simulink model "planta_codesys_opc"  (R2025b)
settings: Solver=FixedStepAuto  StartTime=0.0  StopTime=inf  FixedStep=Ts2  RelTol=1e-3
values from neighbouring files (symbols this model uses):
  ah_max = 0.75    [init_plant_parameters.m]
  at_max = 0.80    (= 0.8)    [init_plant_parameters.m]
  bcx = 1.0e6    (= 1000000)    [init_plant_parameters.m]
  bcy = 10.0e6    (= 10000000)    [init_plant_parameters.m]
  bh_eq = bhm+bhd/ih^2    (= 18.0165289256)    [init_plant_parameters.m]
  bhb = 100e6    (= 100000000)    [init_plant_parameters.m]
  bhEb = 2.2e9    (= 2200000000)    [init_plant_parameters.m]
  bhwu = 150    [init_plant_parameters.m]
  bt = 90.0    (= 90)    [init_plant_parameters.m]
  bt_eq = btm+btd/it^2    (= 6.002)    [init_plant_parameters.m]
  btb = 5.0e6    (= 5000000)    [init_plant_parameters.m]
  btw = 3.0e3    (= 3000)    [init_plant_parameters.m]
  g = 9.80665    [init_plant_parameters.m]
  Hc = 2.59    [init_plant_parameters.m]
  ih = 22.0    (= 22)    [init_plant_parameters.m]
  it = 30.0    (= 30)    [init_plant_parameters.m]
  Jh_eq = Jhm_hb+Jhd_hEb/ih^2    (= 37.8512396694)    [init_plant_parameters.m]
  Jt_eq = Jtm_tb+Jtd/it^2    (= 8.33333333333)    [init_plant_parameters.m]
  k_i_c = abs(polos_obs_c)^3    [init_plant_parameters.m]
  k_i_h = abs(polos_obs_h)^3    [init_plant_parameters.m]
  k_omega_c = 3 * abs(polos_obs_c)^2    [init_plant_parameters.m]
  k_omega_h = 3 * abs(polos_obs_h)^2-k_tita_h*bh_eq/Jh_eq    [init_plant_parameters.m]
  k_tita_c = 3 * abs(polos_obs_c)    [init_plant_parameters.m]
  k_tita_h = 3 * abs(polos_obs_h)-bh_eq/Jh_eq    [init_plant_parameters.m]
  Kcy = 1.8e9    (= 1800000000)    [init_plant_parameters.m]
  khwu = 236e6    (= 236000000)    [init_plant_parameters.m]
  Ki_c = (wn_t^2*Mt)/Kf    (= 320)    [init_plant_parameters.m]
  Ki_i = (wn_h^2)*Jh_eq    (= 2422.47933884)    [init_plant_parameters.m]
  Kp_c = (2*zitta_t*wn_t*Mt)/Kf    (= 1120)    [init_plant_parameters.m]
  Kp_i = 2*zitta_h*wn_h*Jh_eq    (= 1211.23966942)    [init_plant_parameters.m]
  Ktw = 480e3    (= 480000)    [init_plant_parameters.m]
  Lh0 = 110    [init_plant_parameters.m]
  lh_0 = Yt0-yh_0    (= 7)    [init_plant_parameters.m]
  Mc_max = 50000    [init_plant_parameters.m]
  Mc_min = 2000    [init_plant_parameters.m]
  Ms = 15000    [init_plant_parameters.m]
  Mt = 30000    [init_plant_parameters.m]
  rhd = 0.75    [init_plant_parameters.m]
  rtd = 0.50    (= 0.5)    [init_plant_parameters.m]
  tau_hm = Ts2    (= 0.001)    [init_plant_parameters.m]
  tau_tm = Ts2    (= 0.001)    [init_plant_parameters.m]
  Thb_Max = 50e3    (= 50000)    [init_plant_parameters.m]
  ThEb_Max = 1.1e6    (= 1100000)    [init_plant_parameters.m]
  Thm_0 = 0    [init_plant_parameters.m]
  Thm_Max = 20e3    (= 20000)    [init_plant_parameters.m]
  titahm_0 = yl_0/(rhd/(2*ih))    (= 2228.19975108)    [init_plant_parameters.m]
  titatm_0 = xtd_0/(rtd/it)    (= 300)    [init_plant_parameters.m]
  Ts0 = 0.02    [init_plant_parameters.m]
  Ts1 = 0.02    [init_plant_parameters.m]
  Ttb_Max = 5.0e3    (= 5000)    [init_plant_parameters.m]
  Ttm_0 = 0    [init_plant_parameters.m]
  Ttm_Max = 4.0e3    (= 4000)    [init_plant_parameters.m]
  vh_0 = 0    [init_plant_parameters.m]
  vh_max = 3    [init_plant_parameters.m]
  vh_nom = 1.5    [init_plant_parameters.m]
  vt_0 = 0    [init_plant_parameters.m]
  vt_max = 4.0    (= 4)    [init_plant_parameters.m]
  Wc = 2.44    [init_plant_parameters.m]
  xl_0 = 5    [init_plant_parameters.m]
  xt_0 = 5    [init_plant_parameters.m]
  xt_max = 50.0    (= 50)    [init_plant_parameters.m]
  xt_min = -30.0    (= -30)    [init_plant_parameters.m]
  xtd_0 = xt_0    (= 5)    [init_plant_parameters.m]
  yh_max = 40    [init_plant_parameters.m]
  yh_min = -20    [init_plant_parameters.m]
  yl_0 = Yt0 - l_0    (= 37.9806775752)    [init_plant_parameters.m]
  Yt0 = 45.0    (= 45)    [init_plant_parameters.m]
  zitta = 0.5    [init_plant_parameters.m]
undefined symbols (not defined in the file or in its folder): DiscIntNeverNeededParam
libraries: opcualib x6, sl3dlib x1, simulink_extras x1, dspnetwork x1
(part 2 of 2)

== system planta_codesys_opc/Subsystem2/Observador de estado ==
  Ttm_ref : Inport
  tita_tm_enc : Inport  Port=2
  Delay One Step1 : Delay  Commented=through  DelayLength=1  InitialCondition=xtd_0
  Discrete-Time Integrator : DiscreteIntegrator  SampleTime=-1  ICPrevOutput=DiscIntNeverNeededParam  ICPrevScaledInput=DiscIntNeverNeededParam
  Discrete-Time Integrator1 : DiscreteIntegrator  InitialCondition=titatm_0  SampleTime=-1  ICPrevOutput=DiscIntNeverNeededParam  ICPrevScaledInput=DiscIntNeverNeededParam
  Discrete-Time Integrator2 : DiscreteIntegrator  SampleTime=-1  ICPrevOutput=DiscIntNeverNeededParam  ICPrevScaledInput=DiscIntNeverNeededParam
  Gain : Gain  Gain=1/Jt_eq
  Gain1 : Gain  Gain=k_omega_c
  Gain2 : Gain  Gain=k_tita_c
  Gain3 : Gain  Gain=k_i_c
  Gain4 : Gain  Gain=rtd/it
  Sum4 : Sum  Inputs=|++
  Sum5 : Sum  Inputs=|++
  Sum6 : Sum  Inputs=+-|
  Sum7 : Sum  Inputs=|++
  vt_obs : Outport
  wires:
  Discrete-Time Integrator/1 -> Sum5/1
  Sum4/1 -> Discrete-Time Integrator/1
  tita_tm_enc/1 -> Delay One Step1/1
  Discrete-Time Integrator2/1 -> Gain3/1
  Gain1/1 -> Sum4/2
  Sum6/1 -> Discrete-Time Integrator2/1, Gain1/1, Gain2/1
  Discrete-Time Integrator1/1 -> Sum6/2
  Sum7/1 -> Sum4/1
  Gain3/1 -> Sum7/2
  Gain/1 -> Sum7/1
  Gain2/1 -> Sum5/2
  Ttm_ref/1 -> Gain/1
  Sum5/1 -> Gain4/1, Discrete-Time Integrator1/1
  Delay One Step1/1 -> Sum6/1
  Gain4/1 -> vt_obs/1

== system planta_codesys_opc/Subsystem/Carro/Subsystem ==
  BRK_t : Inport
  w_tm : Inport  Port=2
  Constant : Constant  Value=0
  Gain1 : Gain  Gain=-Ttb_Max
  Gain8 : Gain  Gain=btb
  Switch : Switch  Criteria=u2 > Threshold  SaturateOnIntegerOverflow=off  InputSameDT=off
  Tanh : Trigonometry  Operator=tanh
  T_tb : Outport
  wires:
  Constant/1 -> Switch/1
  BRK_t/1 -> Switch/2
  Switch/1 -> T_tb/1  "T_tb"
  w_tm/1 -> Gain8/1
  Gain8/1 -> Tanh/1
  Tanh/1 -> Gain1/1
  Gain1/1 -> Switch/3

== system planta_codesys_opc/Subsystem/Subsystem2/Subsystem ==
  T_tm* : Inport
  Constant : Constant  Value=Ttm_Max
  Constant1 : Constant  Value=-Ttm_Max
  Gain : Gain  Gain=1/tau_tm
  Integrator : Integrator
  Max : MinMax  Function=max  Inputs=2
  Min : MinMax  Inputs=2
  Sum : Sum  Inputs=|+-
  Zero-Order Hold : ZeroOrderHold  SampleTime=tau_tm
  T_tm : Outport
  wires:
  Min/1 -> Sum/1
  Gain/1 -> Integrator/1
  Sum/1 -> Gain/1
  Integrator/1 -> Sum/2, T_tm/1
  Max/1 -> Min/2
  Constant/1 -> Min/1
  Constant1/1 -> Max/1
  T_tm*/1 -> Zero-Order Hold/1
  Zero-Order Hold/1 -> Max/2

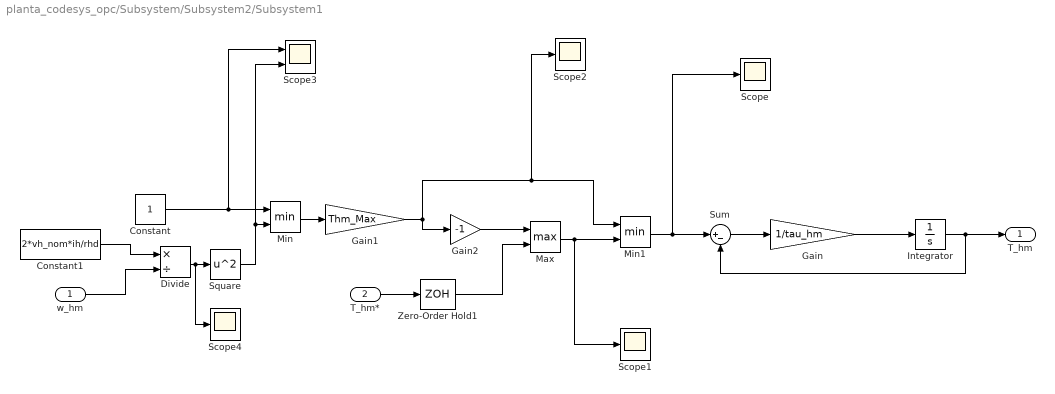
== system planta_codesys_opc/Subsystem/Subsystem2/Subsystem1 ==
  w_hm : Inport
  T_hm* : Inport  Port=2
  Constant : Constant
  Constant1 : Constant  Value=2*vh_nom*ih/rhd
  Divide : Product  Inputs=*/
  Gain : Gain  Gain=1/tau_hm
  Gain1 : Gain  Gain=Thm_Max
  Gain2 : Gain  Gain=-1
  Integrator : Integrator
  Max : MinMax  Function=max  Inputs=2
  Min : MinMax  Inputs=2
  Min1 : MinMax  Inputs=2
  Scope{,1..2,4} (4 alike) : Scope
      Scope settings: ActiveDisplayYMinimum=-2500  ActiveDisplayYMaximum=22500  DataLoggingVariableName=ScopeData3
      Scope1 settings: ActiveDisplayYMinimum=-2500  ActiveDisplayYMaximum=22500  DataLoggingVariableName=ScopeData4
      Scope2 settings: ActiveDisplayYMinimum=481.45655  ActiveDisplayYMaximum=22168.72705  DataLoggingVariableName=ScopeData5
      Scope4 settings: ActiveDisplayYMinimum=-0.06596  ActiveDisplayYMaximum=-0.00953  DataLoggingVariableName=ScopeData7
  Scope3 : Scope  NumInputPorts=2
      settings: ActiveDisplayYMinimum=-9.1717430786370772E+28  ActiveDisplayYMaximum=8.25456877077337E+29  DataLoggingVariableName=ScopeData6
  Square : Math  Operator=square
  Sum : Sum  Inputs=|+-
  Zero-Order Hold1 : ZeroOrderHold  SampleTime=tau_hm
  T_hm : Outport
  wires:
  Sum/1 -> Gain/1
  Gain/1 -> Integrator/1
  Integrator/1 -> Sum/2, T_hm/1
  Constant/1 -> Scope3/1, Min/1
  w_hm/1 -> Divide/2
  Constant1/1 -> Divide/1
  Divide/1 -> Scope4/1, Square/1
  Square/1 -> Scope3/2, Min/2
  Min/1 -> Gain1/1
  Gain1/1 -> Scope2/1, Min1/1, Gain2/1
  T_hm*/1 -> Zero-Order Hold1/1
  Gain2/1 -> Max/1
  Max/1 -> Scope1/1, Min1/2
  Min1/1 -> Scope/1, Sum/1
  Zero-Order Hold1/1 -> Max/2

== system planta_codesys_opc/Subsystem/accionamiento izaje/brake izaje ==
  w_hm : Inport
  BRK_h : Inport  Port=2
  Constant : Constant  Value=0
  Gain : Gain  Gain=bhb
  Gain1 : Gain  Gain=-Thb_Max
  Switch : Switch  Criteria=u2 > Threshold  SaturateOnIntegerOverflow=off  InputSameDT=off
  Tanh : Trigonometry  Operator=tanh
  T_hb : Outport
  wires:
  Switch/1 -> T_hb/1
  Constant/1 -> Switch/1
  BRK_h/1 -> Switch/2
  w_hm/1 -> Gain/1
  Gain/1 -> Tanh/1
  Tanh/1 -> Gain1/1
  Gain1/1 -> Switch/3

== system planta_codesys_opc/Subsystem/accionamiento izaje/brake izaje emergencia ==
  w_hd : Inport
  BRK_hE : Inport  Port=2
  Constant : Constant  Value=0
  Gain : Gain  Gain=bhEb
  Gain1 : Gain  Gain=-ThEb_Max
  Switch : Switch  Criteria=u2 > Threshold  SaturateOnIntegerOverflow=off  InputSameDT=off
  Tanh : Trigonometry  Operator=tanh
  T_hEb : Outport
  wires:
  Tanh/1 -> Gain1/1
  Gain/1 -> Tanh/1
  Constant/1 -> Switch/1
  w_hd/1 -> Gain/1
  Switch/1 -> T_hEb/1
  BRK_hE/1 -> Switch/2
  Gain1/1 -> Switch/3

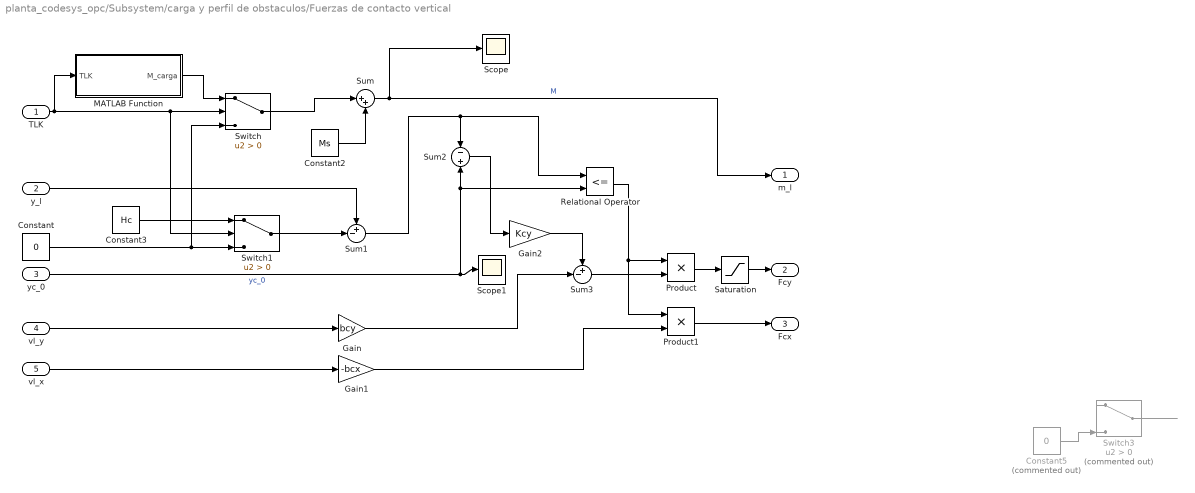
== system planta_codesys_opc/Subsystem/carga y perfil de obstaculos/Fuerzas de contacto vertical ==
  TLK : Inport
  y_l : Inport  Port=2
  yc_0 : Inport  Port=3
  vl_y : Inport  Port=4
  vl_x : Inport  Port=5
  Constant : Constant  Value=0
  Constant2 : Constant  Value=Ms
  Constant3 : Constant  Value=Hc
  Constant5 : Constant  Commented=on  Value=0
  Gain : Gain  Gain=bcy
  Gain1 : Gain  Gain=-bcx
  Gain2 : Gain  Gain=Kcy
  MATLAB Function : MATLAB Function  TreatAsAtomicUnit=on
  Product : Product
  Product1 : Product
  Relational Operator : RelationalOperator  Operator=<=  OutDataTypeStr=boolean  RndMeth=Simplest  InputSameDT=off
  Saturation : Saturate  UpperLimit=inf  LowerLimit=0
  Scope : Scope
      settings: ActiveDisplayYMinimum=-30040.049311756404  ActiveDisplayYMaximum=65258.780060315854  DataLoggingVariableName=ScopeData31
  Scope1 : Scope
      settings: ActiveDisplayYMinimum=12.776564460216019  ActiveDisplayYMaximum=15.5369149188378  DataLoggingVariableName=ScopeData32
  Sum : Sum  Inputs=|++
  Sum1 : Sum  Inputs=+-|
  Sum2 : Sum  Inputs=-|+
  Sum3 : Sum  Inputs=+-|
  Switch : Switch  Criteria=u2 > Threshold  SaturateOnIntegerOverflow=off  InputSameDT=off
  Switch1 : Switch  Criteria=u2 > Threshold  SaturateOnIntegerOverflow=off  InputSameDT=off
  Switch3 : Switch  Commented=on  Criteria=u2 > Threshold  SaturateOnIntegerOverflow=off  InputSameDT=off
  m_l : Outport
  Fcy : Outport  Port=2
  Fcx : Outport  Port=3
  wires:
  MATLAB Function/1(M_carga) -> Switch/1
  TLK/1 -> MATLAB Function/1(TLK), Switch1/2, Switch/2
  Constant/1 -> Switch1/3, Switch/3
  Constant3/1 -> Switch1/1
  Switch/1 -> Sum/1
  Sum/1 -> Scope/1, m_l/1  "M"
  Constant2/1 -> Sum/2
  Switch1/1 -> Sum1/2
  y_l/1 -> Sum1/1
  Sum1/1 -> Relational Operator/1, Sum2/1
  yc_0/1 -> Scope1/1, Sum2/2, Relational Operator/2  "yc_0"
  Sum2/1 -> Gain2/1
  Gain2/1 -> Sum3/1
  Relational Operator/1 -> Product1/1, Product/1
  Product1/1 -> Fcx/1
  Gain/1 -> Sum3/2
  vl_y/1 -> Gain/1
  vl_x/1 -> Gain1/1
  Gain1/1 -> Product1/2
  Sum3/1 -> Product/2
  Constant5/1 -> Switch3/3
  Switch3/1 -> ?
  ? -> Switch3/1, Switch3/2
  Product/1 -> Saturation/1
  Saturation/1 -> Fcy/1

== matlab function planta_codesys_opc/Subsystem/carga y perfil de obstaculos/MATLAB Function ==
  data: y0_array input; yc0_xt output; index input
function yc0_xt= calcula_y0(y0_array,index)
index = floor(index)+1;
index = min(max(index,1),33);
yc0_xt = y0_array(index);

== matlab function planta_codesys_opc/Subsystem/carga y perfil de obstaculos/Fuerzas de contacto vertical/MATLAB Function ==
  settings: updateMethod=DISCRETE
  data: TLK input; M_carga output; Mc_min parameter; Mc_max parameter
function M_carga = Masa_Aleatoria(TLK, Mc_min, Mc_max)
    persistent masa_actual;
    persistent ultimo_estado_trigger;
    
    % Inicialización
    if isempty(masa_actual)
        masa_actual = Mc_min; % Empezamos con el valor mínimo por defecto
        ultimo_estado_trigger = 0;
    end
    
    % DETECCIÓN DE FLANCO DE SUBIDA (Rising Edge)
    if (TLK == 1 && ultimo_estado_trigger == 0)
        % Generar carga aleatoria entre 3tn y 55tn (para tener sobrecarga)
        masa_actual = Mc_min + (Mc_max + 5000 - Mc_min) * rand();
        masa_actual = round(masa_actual); 
    end
    
    % Actualizar memoria del trigger
    ultimo_estado_trigger = TLK;
    % Salida: La masa se mantiene constante hasta el próximo trigger
    M_carga = masa_actual;
end

== matlab function planta_codesys_opc/Control Joystick /MATLAB Function ==
  data: BTN input; BTN_re output
function BTN_re = fcn(BTN)
    persistent prev;
    persistent state;
    if isempty(prev)
        prev = 0;
        state = 0;
    end
    if BTN == 1 && prev == 0
        state = double(~logical(state));
    end
    BTN_re = state;
    prev = double(BTN);
end
